simulink model "DroneModel"  (R2026b)
settings: Solver=VariableStepAuto
settings Model: Creator=y6753  LastModifiedBy=y6753
settings SimscapeCC: SimscapeLogType=all  SimscapeNominalValues="[{\"value\":\"1\",\"unit\":\"A\"},{\"value\":\"1\",\"unit\":\"bar\"},{\"value\":\"1\",\"unit\":\"cm^2\"},{\"value\":\"1\",\"unit\":\"cm^3/s\"},{\"value\":\"1\",\"unit\":\"kJ/kg\"},{\"value\":\"1\",\"unit\":\"kW\"},{\"value\":\"1\",\"unit\":\"l\"},{\"value\":\"1\",\"unit\":\"N\"},{\"value\":\"1\",\"unit\":\"N*m\"},{\"value\":\"1\",\"unit\":\"V\"},{\"value\":\"0.001\",\"unit\":\"Wb\"}]"  SimscapeUseEnergyAccounting=off

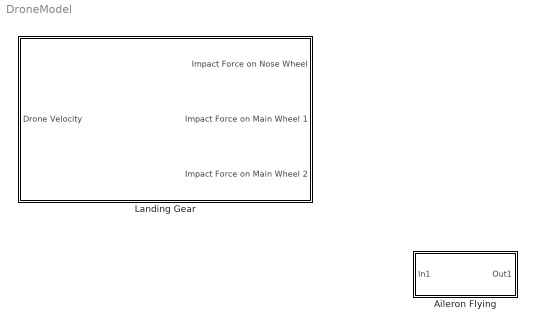
== system DroneModel ==
  Aileron Flying : Subsystem
  Landing Gear : Subsystem

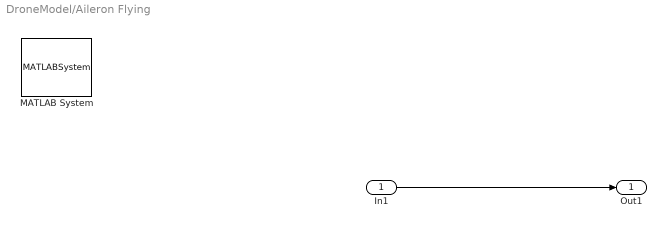
== system DroneModel/Aileron Flying ==
  In1 : Inport
  MATLAB System : MATLABSystem
  Out1 : Outport
  wires:
  In1/1 -> Out1/1

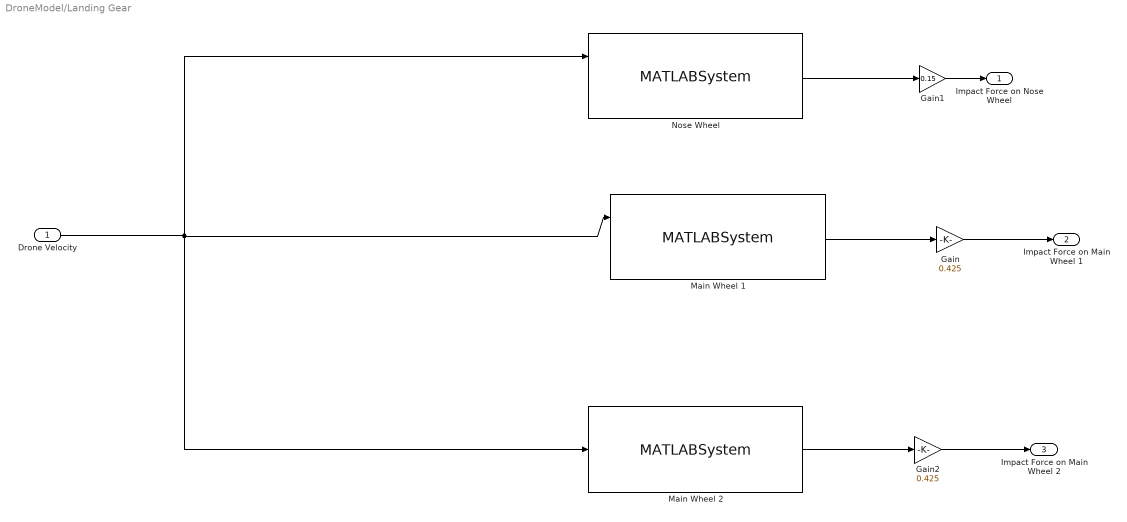
== system DroneModel/Landing Gear ==
  Drone Velocity : Inport
  Gain : Gain  Gain=0.425
  Gain1 : Gain  Gain=0.15
  Gain2 : Gain  Gain=0.425
  Main Wheel 1 : MATLABSystem  System=Wheel_Force  drone_mass=4.25  SimulateUsing=Code generation
      mask Type: Wheel_Force
  Main Wheel 2 : MATLABSystem  System=Wheel_Force  drone_mass=4.25  vert_dist=1  SimulateUsing=Code generation
      mask Type: Wheel_Force
  Nose Wheel : MATLABSystem  System=Wheel_Force  drone_mass=4.25  SimulateUsing=Code generation
      mask Type: Wheel_Force
  Impact Force on Nose Wheel : Outport
  Impact Force on Main Wheel 1 : Outport  Port=2
  Impact Force on Main Wheel 2 : Outport  Port=3
  wires:
  Drone Velocity/1 -> Nose Wheel/1, Main Wheel 1/1, Main Wheel 2/1
  Nose Wheel/1 -> Gain1/1
  Main Wheel 1/1 -> Gain/1
  Gain/1 -> Impact Force on Main Wheel 1/1
  Gain1/1 -> Impact Force on Nose Wheel/1
  Main Wheel 2/1 -> Gain2/1
  Gain2/1 -> Impact Force on Main Wheel 2/1
